simulink model "sf_backup_undesirable"  (R2025b)
settings: Solver=FixedStepDiscrete  StartTime=0.0  StopTime=1  FixedStep=.2  RelTol=1e-3  EnableMultiTasking=on
settings Model: Creator=The MathWorks, Inc.  LastModifiedBy=The MathWorks, Inc.
settings SolverCC: AlgebraicLoopSolver=TrustRegion  MaxZcPerStep=1.0
settings DataIOCC: LimitDataPoints=on  SaveFormat=Array  ReturnWorkspaceOutputs=off
settings OptimizationCC: ReuseModelBlockBuffer=off  ExpressionDepthLimit=2147483647.0  InitFltsAndDblsToZero=on  LifeSpan=inf
settings DebuggingCC: SaveWithParameterizedLinksMsg=none  UnderspecifiedInitializationDetection=Classic  MergeDetectMultiDrivingBlocksExec=none  SignalResolutionControl=TryResolveAllWithWarning  SolverPrmCheckMsg=warning  MultiTaskDSMMsg=warning  MultiTaskCondExecSysMsg=none  FcnCallInpInsideContextMsg=warning  UnconnectedInputMsg=warning  UnconnectedOutputMsg=warning  UnconnectedLineMsg=warning  StateNameClashWarn=warning  SFUnexpectedBacktrackingDiag=warning  SFNoUnconditionalDefaultTransitionDiag=warning  SFExecutionAtInitializationDiag=none  ArithmeticOperatorsInVariantConditions=warning
settings HardwareCC: ProdBitPerPointer=32.0  ProdBitPerSizeT=32.0  ProdBitPerPtrDiffT=32.0  ProdLargestAtomicFloat=None  ProdIntDivRoundTo=Undefined  ProdEndianess=Unspecified  ProdWordSize=32.0  ProdHWDeviceType=32-bit Generic
settings ModelReferenceCC: EnableRefExpFcnMdlSchedulingChecks=on  PropagateSignalLabelsOutOfModel=off
settings SFSimCC: SimUseLocalCustomCode=off  SimParseCustomCode=off  CustomCodeUndefinedFunction=UseInterfaceOnly
settings RTWCC: RTWUseLocalCustomCode=off  GPUComputeCapability=3.5  DLArmComputeVersion=19.05
settings CodeAppCC: StateflowObjectComments=on
settings GRTTargetCC: TargetFcnLib=ansi_tfl_tmw.mat  TargetLangStandard=C89/C90 (ANSI)  CombineOutputUpdateFcns=off  GRTInterface=on
settings ConfigComp: CovMetricSettings=dw  CovSaveCumulativeToWorkspaceVar=on  CovSaveSingleToWorkspaceVar=on  CovExternalEMLEnable=off  CovSFcnEnable=off

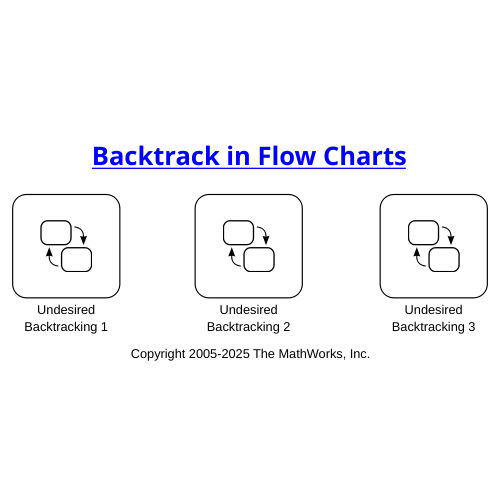
[thumbnail: Simulink's stored preview of the top-level diagram]
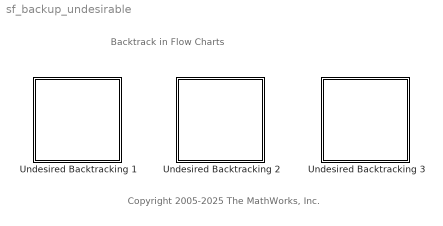
== system sf_backup_undesirable ==
  note: Copyright 2005-2025 The MathWorks, Inc.
  note: Backtrack in Flow Charts
  Undesired Backtracking 1 : Stateflow chart  TreatAsAtomicUnit=on
  Undesired Backtracking 2 : Stateflow chart  TreatAsAtomicUnit=on
      settings: RTWFcnNameOpts=Use subsystem name  RTWFileNameOpts=Use subsystem name
  Undesired Backtracking 3 : Stateflow chart  TreatAsAtomicUnit=on
      settings: RTWFcnNameOpts=Use subsystem name  RTWFileNameOpts=Use subsystem name

== stateflow chart sf_backup_undesirable/Undesired Backtracking 3 ==
  settings: updateMethod=DISCRETE  executeAtInitialization=1
  state BAD [function]
    note: This function shows an example of backtracking semantics that can lead to inefficient run-time behavior. A cursory look at the flow chart might lead you to believe that it represents this logic:
        |
        | if ((c1 || c2) &&
        | (c3 || c4) &&
        | (c5 || c6) &&
        | (c7))
        | {
        | a1;
        | }
        |
        | If all the conditions are true except c7, the backtracking semantics will cause the function to evaluate some conditions multiple times. For example, the function evaluates the condition c6 three times.
    (default) -> (junction 45)
    (junction 45) -> (junction 46) [order 2] : [c2]
    (junction 45) -> (junction 46) [order 1] : [c1]
    (junction 46) -> (junction 47) [order 2] : [c4]
    (junction 46) -> (junction 47) [order 1] : [c3]
    (junction 47) -> (junction 48) [order 2] : [c6]
    (junction 47) -> (junction 48) [order 1] : [c5]
    (junction 48) -> (junction 50) : [c7]{a1;}
  state GOOD [function]
    note: In this function, a transition to a terminal junction prevents the undesired backtracking, so each condition is evaluated only once.
    (default) -> (junction 78)
    (junction 78) -> (junction 81) [order 2] : [c2]
    (junction 78) -> (junction 81) [order 1] : [c1]
    (junction 81) -> (junction 79) [order 2] : [c4]
    (junction 81) -> (junction 79) [order 1] : [c3]
    (junction 79) -> (junction 80) [order 2] : [c6]
    (junction 79) -> (junction 80) [order 1] : [c5]
    (junction 80) -> (junction 91) [order 2]
    (junction 80) -> (junction 83) [order 1] : [c7]{a1;}
  data: a1 local double; c1 local double; c2 local double; c3 local double; c4 local double; c5 local double; c6 local double; c7 local double

== stateflow chart sf_backup_undesirable/Undesired Backtracking 1 ==
  state GOOD [function]
    note: In this function, there are no junctions with multiple incoming paths. This design pattern prevents backtracking, so the function increments the local variable x exactly once.
    (default) -> (junction 48)
    (junction 48) -> (junction 49) : [c1 || c2]
    (junction 49) -> (junction 50) : [c3]{x++;}
    (junction 50) -> (junction 51) : [c4]
  state BAD [function]
    note: This function shows an example of backtracking semantics that may not be expected or desired. When conditions c1, c2, and c3 are true and c4 is false, the backtracking semantics increment the local data x multiple times.
        |
        | 1. The function determines that c1 is true.
        | 2. The function determines that c3 is true, so it increments x.
        | 3. The function determines that c4 is false, so the execution backtracks to the last junction which still has unevaluated transitions.
        | 4. The function determines that c2 is true.
        | 5. The function determines that c3 is true, so it increments x again.
        | 6. The function determines that c4 is false. This time there are no transitions to backtrack to so execution stops.
    (default) -> (junction 38)
    (junction 38) -> (junction 39) [order 1] : [c2]
    (junction 38) -> (junction 39) [order 2] : [c1]
    (junction 39) -> (junction 43) : [c3]{x++;}
    (junction 43) -> (junction 45) : [c4]
  data: x local double; c1 local double =1; c2 local double; c3 local double =0; c4 local double

== stateflow chart sf_backup_undesirable/Undesired Backtracking 2 ==
  settings: updateMethod=DISCRETE  executeAtInitialization=1
  state BAD [function]
    note: This function shows an example of backtracking semantics that may not be expected or desired. A cursory look at the flow chart might lead you to believe that it represents this logic:
        |
        | if (c1) {
        | a1;
        | } else {
        | a2;
        | }
        |
        | if (c2) {
        | a3;
        | }
        |
        | However, when c1 is true but c2 is false, backtracking
        | semantics execute both of the actions a1 and a2. After the function executes a2, the function evaluates c2 as false. Then, the function backtracks to the transition that was not previously evaluated and executes a2.
    (default) -> (junction 9)
    (junction 9) -> (junction 14) [order 1] : [c1]
    (junction 14) -> (junction 15) : {a2;}
    (junction 9) -> (junction 10) [order 2] : {a1;}
    (junction 15) -> (junction 10)
    (junction 10) -> (junction 11)
    (junction 11) -> (junction 13) : [c2]
    (junction 13) -> (junction 12) : {a3;}
  state GOOD [function]
    note: This function avoids the problem of undesired backtracking by adding a transition to a second terminal junction. This transition prevents the function from backtracking. When the function evaluates c2 as false, it executes the transition to the terminal junction and stops.
    (default) -> (junction 23)
    (junction 23) -> (junction 24) [order 1] : [c1]
    (junction 24) -> (junction 26) : {a2;}
    (junction 23) -> (junction 25) [order 2] : {a1;}
    (junction 26) -> (junction 25)
    (junction 25) -> (junction 27)
    (junction 27) -> (junction 28) [order 1] : [c2]
    (junction 27) -> (junction 40) [order 2]
    (junction 28) -> (junction 29) : {a3;}
  data: a1 local double; a2 local double; a3 local double; c1 local double; c2 local double
